simulink subsystem "Actuators_TVC_RCS"  (R2026a)
settings: Solver=VariableStepAuto
undefined symbols (not defined in the file): ENGINE, IN, VEH
libraries: simulink_extras x4, matrix_library x1
settings Model: Creator=asing  LastModifiedBy=asing

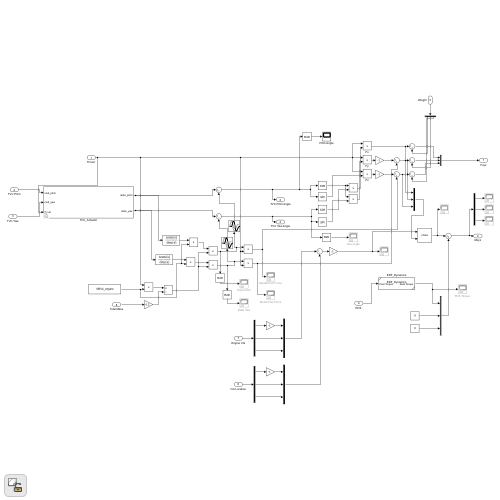
[thumbnail: Simulink's stored preview of the top-level diagram]
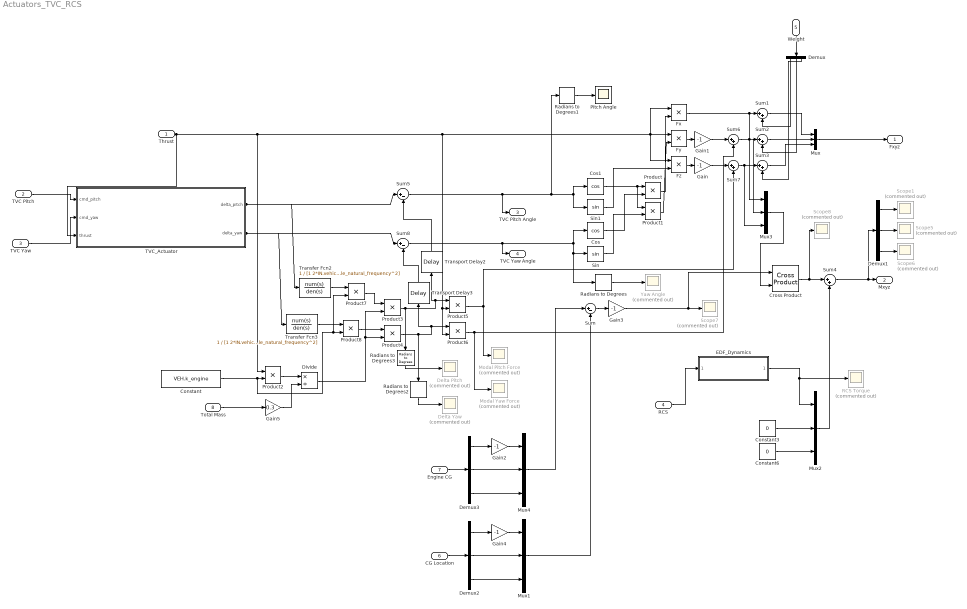
== system Actuators_TVC_RCS ==
  "Thrust " : Inport
  TVC Pitch : Inport  Port=2
  TVC Yaw : Inport  Port=3
  "RCS " : Inport  Port=4
  Weight : Inport  Port=5
  CG Location : Inport  Port=6
  Engine CG : Inport  Port=7
  Total Mass : Inport  Port=8
  Constant : Constant  Value=VEH.k_engine
  Constant3 : Constant  Value=0
  Constant6 : Constant  Value=0
  Cos : Trigonometry  Operator=cos
  Cos1 : Trigonometry  Operator=cos
  Cross Product : matrix_library/Cross Product
  Delta Pitch : Scope  Commented=on
      settings: ActiveDisplayYMinimum=-0.0038016775387335047  ActiveDisplayYMaximum=0.0038576393364572227  DataLoggingVariableName=ScopeData83
  Delta Yaw : Scope  Commented=on
      settings: ActiveDisplayYMinimum=-0.0018754271280055322  ActiveDisplayYMaximum=0.0029155281667496203  DataLoggingVariableName=ScopeData84
  Demux{,1..3} (4 alike) : Demux  Outputs=3
  Divide : Product  Inputs=*/
  EDF_Dynamics : Subsystem  ReferencedSubsystem=EDF_Dynamics
  Fx : Product
  Fy : Product
  Fz : Product
  Gain{,1..4} (5 alike) : Gain  Gain=-1
  Gain5 : Gain  Gain=0.3
  Modal Pitch Force : Scope  Commented=on
      settings: ActiveDisplayYMinimum=-0.088739631277941974  ActiveDisplayYMaximum=0.086025104693778914  DataLoggingVariableName=ScopeData78
  Modal Yaw Force : Scope  Commented=on
      settings: ActiveDisplayYMinimum=-0.017420268895536287  ActiveDisplayYMaximum=0.028077380315148965  DataLoggingVariableName=ScopeData79
  Mux{,1..4} (5 alike) : Mux  Inputs=3
  Pitch Angle : Scope
      settings: ActiveDisplayYMinimum=-10.903439073445846  ActiveDisplayYMaximum=7.4616563198748231  DataLoggingVariableName=ScopeData71
  Product{,1..8} (9 alike) : Product
  RCS Torque : Scope  Commented=on
      settings: ActiveDisplayYMinimum=-8.021209014289818  ActiveDisplayYMaximum=10.60123996530198  DataLoggingVariableName=ScopeData47
  Radians to Degrees{,1..3} (4 alike) : simulink_extras/Transformations/Radians to Degrees
  Scope{1,5..8} (5 alike) : Scope  Commented=on
      Scope1 settings: ActiveDisplayYMinimum=0.090000000000000011  ActiveDisplayYMaximum=0.11  DataLoggingVariableName=ScopeData50
      Scope5 settings: ActiveDisplayYMinimum=-1  ActiveDisplayYMaximum=1  DataLoggingVariableName=ScopeData54
      Scope6 settings: ActiveDisplayYMinimum=-1  ActiveDisplayYMaximum=1  DataLoggingVariableName=ScopeData55
      Scope7 settings: ActiveDisplayYMinimum=-1.008334185713273  ActiveDisplayYMaximum=-0.924758879501166  DataLoggingVariableName=ScopeData56
      Scope8 settings: ActiveDisplayYMinimum=-1  ActiveDisplayYMaximum=1  DataLoggingVariableName=ScopeData60
  Sin : Trigonometry
  Sin1 : Trigonometry
  Sum : Sum  Inputs=|+-
  Sum{1..4,6..7} (6 alike) : Sum  Inputs=|++
  Sum5 : Sum  Inputs=|+-
  Sum8 : Sum  Inputs=|+-
  TVC_Actuator : Subsystem  Variant=on
  Transfer Fcn2 : TransferFcn  Numerator=1  Denominator=[1 2*IN.vehicle_damping_ratio*IN.vehicle_natural_frequency IN.vehicle_natural_frequency^2]
  Transfer Fcn3 : TransferFcn  Numerator=1  Denominator=[1 2*IN.vehicle_damping_ratio*IN.vehicle_natural_frequency IN.vehicle_natural_frequency^2]
  Transport Delay2 : TransportDelay  DelayTime=0.01
  Transport Delay3 : TransportDelay  DelayTime=0.01
  Yaw Angle : Scope  Commented=on
      settings: ActiveDisplayYMinimum=-1.8231379337691429  ActiveDisplayYMaximum=5.2718467554145434  DataLoggingVariableName=ScopeData70
  Fxyz : Outport
  Mxyz : Outport  Port=2
  TVC Pitch Angle : Outport  Port=3
  TVC Yaw Angle : Outport  Port=4
  wires:
  Cos1/1 -> Product/1, Product1/1
  Cos/1 -> Product/2
  Product/1 -> Fx/2
  "Thrust "/1 -> Fz/1, Fy/1, Fx/1, Product5/2, Product6/2, Product2/1, TVC_Actuator/3(thrust)
  Mux/1 -> Fxyz/1
  Sum1/1 -> Mux/1
  Weight/1 -> Demux/1
  Fy/1 -> Gain1/1
  Sum2/1 -> Mux/2
  Fz/1 -> Gain/1
  Demux/2 -> Sum2/2
  Mux1/1 -> Sum/2
  Sum/1 -> Gain3/1
  Cross Product/1 -> Sum4/1, Scope8/1
  Constant3/1 -> Mux2/2
  Mux2/1 -> Sum4/2
  Sum4/1 -> Mxyz/1, Demux1/1
  Demux1/1 -> Scope1/1
  Demux1/2 -> Scope5/1
  Demux1/3 -> Scope6/1
  Product1/1 -> Fy/2
  Sin/1 -> Product1/2
  Sin1/1 -> Fz/2
  Gain3/1 -> Scope7/1, Cross Product/1
  Sum3/1 -> Mux/3
  Mux3/1 -> Cross Product/2
  Constant6/1 -> Mux2/3
  Demux/1 -> Sum1/2
  Demux/3 -> Sum3/2
  Radians to Degrees/1 -> Yaw Angle/1
  Radians to Degrees1/1 -> Pitch Angle/1
  "RCS "/1 -> EDF_Dynamics/1
  Demux2/3 -> Mux1/3
  CG Location/1 -> Demux2/1
  Demux2/2 -> Mux1/2
  Demux2/1 -> Gain4/1
  Gain4/1 -> Mux1/1
  Gain2/1 -> Mux4/1
  Demux3/1 -> Gain2/1
  Demux3/2 -> Mux4/2
  Demux3/3 -> Mux4/3
  Engine CG/1 -> Demux3/1
  Mux4/1 -> Sum/1
  Total Mass/1 -> Gain5/1
  Product2/1 -> Divide/1
  Gain5/1 -> Divide/2
  Constant/1 -> Product2/2, Product8/2, Product7/2
  Divide/1 -> Product4/2, Product3/2
  Product3/1 -> Radians to Degrees3/1, Product5/1, Transport Delay2/1
  Product4/1 -> Product6/1, Transport Delay3/1, Radians to Degrees2/1
  Fx/1 -> Sum1/1, Mux3/1
  Gain1/1 -> Sum6/1
  Sum6/1 -> Sum2/1, Mux3/2
  Gain/1 -> Sum7/1
  Sum7/1 -> Mux3/3, Sum3/1
  Product5/1 -> Modal Pitch Force/1, Sum7/2
  Product6/1 -> Modal Yaw Force/1, Sum6/2
  Sum5/1 -> Cos1/1, Sin1/1, Radians to Degrees1/1, TVC Pitch Angle/1
  Sum8/1 -> Cos/1, Radians to Degrees/1, Sin/1, TVC Yaw Angle/1
  Radians to Degrees2/1 -> Delta Yaw/1
  Radians to Degrees3/1 -> Delta Pitch/1
  Transport Delay3/1 -> Sum8/2
  Transport Delay2/1 -> Sum5/2
  Transfer Fcn2/1 -> Product7/1
  Product7/1 -> Product3/1
  Transfer Fcn3/1 -> Product8/1
  Product8/1 -> Product4/1
  EDF_Dynamics/1 -> RCS Torque/1, Mux2/1
  TVC Pitch/1 -> TVC_Actuator/1(cmd_pitch)
  TVC Yaw/1 -> TVC_Actuator/2(cmd_yaw)
  TVC_Actuator/1(delta_pitch) -> Sum5/1, Transfer Fcn2/1
  TVC_Actuator/2(delta_yaw) -> Sum8/1, Transfer Fcn3/1

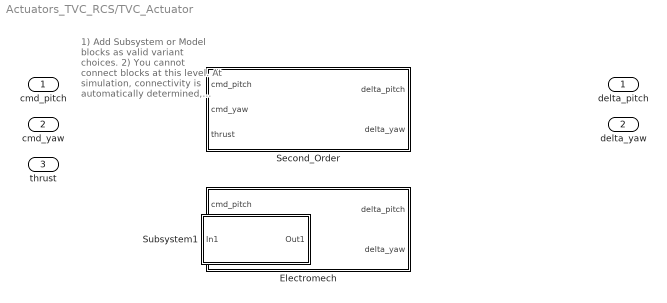
== system Actuators_TVC_RCS/TVC_Actuator ==
  note: 1) Add Subsystem or Model blocks as valid variant choices.
      | 2) You cannot connect blocks at this level. At simulation, connectivity is automatically
      | determined, based on the active variant and port name matching.
  cmd_pitch : Inport
  cmd_yaw : Inport  Port=2
  thrust : Inport  Port=3
  Electromech : Subsystem  VariantControl=VARIANT_TVC_MODEL >= 2
  Second_Order : Subsystem  VariantControl=VARIANT_TVC_MODEL == 1
  Subsystem1 : Subsystem  VariantControl=false
  delta_pitch : Outport
  delta_yaw : Outport  Port=2

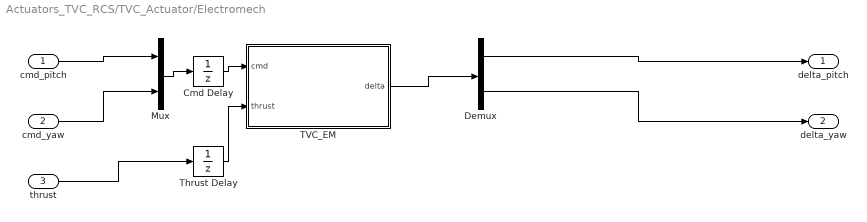
== system Actuators_TVC_RCS/TVC_Actuator/Electromech ==
  cmd_pitch : Inport
  cmd_yaw : Inport  Port=2
  thrust : Inport  Port=3
  Cmd Delay : UnitDelay  SampleTime=1e-3
  Demux : Demux  Outputs=2
  Mux : Mux  Inputs=2
  TVC_EM : MATLAB Function  TreatAsAtomicUnit=on
  Thrust Delay : UnitDelay  SampleTime=1e-3
  delta_pitch : Outport
  delta_yaw : Outport  Port=2
  wires:
  cmd_pitch/1 -> Mux/1
  cmd_yaw/1 -> Mux/2
  Mux/1 -> Cmd Delay/1
  Cmd Delay/1 -> TVC_EM/1(cmd)
  thrust/1 -> Thrust Delay/1
  Thrust Delay/1 -> TVC_EM/2(thrust)
  TVC_EM/1(delta) -> Demux/1
  Demux/1 -> delta_pitch/1
  Demux/2 -> delta_yaw/1

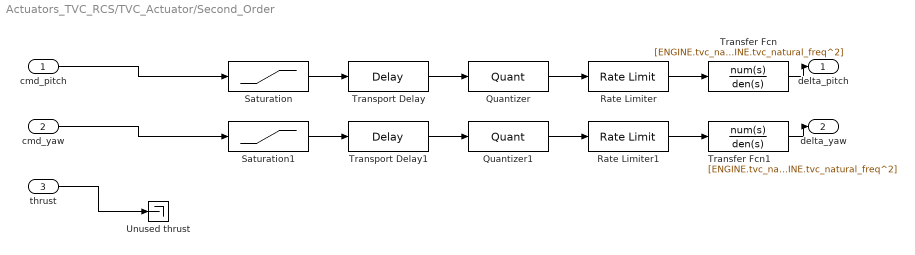
== system Actuators_TVC_RCS/TVC_Actuator/Second_Order ==
  cmd_pitch : Inport
  cmd_yaw : Inport  Port=2
  thrust : Inport  Port=3
  Quantizer : Quantizer  QuantizationInterval=IN.tvc.resolution
  Quantizer1 : Quantizer  QuantizationInterval=IN.tvc.resolution
  Rate Limiter : RateLimiter  RisingSlewLimit=IN.tvc.max_gimbal_rate  FallingSlewLimit=-IN.tvc.max_gimbal_rate  SampleTimeMode=inherited
  Rate Limiter1 : RateLimiter  RisingSlewLimit=IN.tvc.max_gimbal_rate  FallingSlewLimit=-IN.tvc.max_gimbal_rate  SampleTimeMode=inherited
  Saturation : Saturate  UpperLimit=IN.tvc.max_gimbal_angle  LowerLimit=-IN.tvc.max_gimbal_angle
  Saturation1 : Saturate  UpperLimit=IN.tvc.max_gimbal_angle  LowerLimit=-IN.tvc.max_gimbal_angle  LinearizeAsGain=off
  Transfer Fcn : TransferFcn  Numerator=[ENGINE.tvc_natural_freq^2]  Denominator=[1 2*IN.tvc.damping_ratio*ENGINE.tvc_natural_freq ENGINE.tvc_natural_freq^2]
  Transfer Fcn1 : TransferFcn  Numerator=[ENGINE.tvc_natural_freq^2]  Denominator=[1 2*IN.tvc.damping_ratio*ENGINE.tvc_natural_freq ENGINE.tvc_natural_freq^2]
  Transport Delay : TransportDelay  DelayTime=IN.tvc.actuator_latency
  Transport Delay1 : TransportDelay  DelayTime=IN.tvc.actuator_latency
  Unused thrust : Terminator
  delta_pitch : Outport
  delta_yaw : Outport  Port=2
  wires:
  cmd_pitch/1 -> Saturation/1
  Saturation/1 -> Transport Delay/1
  Transport Delay/1 -> Quantizer/1
  Quantizer/1 -> Rate Limiter/1
  Rate Limiter/1 -> Transfer Fcn/1
  Transfer Fcn/1 -> delta_pitch/1
  cmd_yaw/1 -> Saturation1/1
  Saturation1/1 -> Transport Delay1/1
  Transport Delay1/1 -> Quantizer1/1
  Quantizer1/1 -> Rate Limiter1/1
  Rate Limiter1/1 -> Transfer Fcn1/1
  Transfer Fcn1/1 -> delta_yaw/1
  thrust/1 -> Unused thrust/1

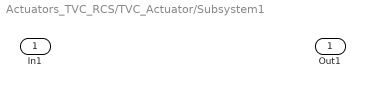
== system Actuators_TVC_RCS/TVC_Actuator/Subsystem1 ==
  In1 : Inport
  Out1 : Outport

== matlab function Actuators_TVC_RCS/TVC_Actuator/Electromech/TVC_EM ==
  data: cmd input; delta output size=[2 1]; thrust input; TVCEM parameter
function delta = TVC_EM(cmd, thrust, TVCEM)
% Erhardt+Leimer TVC actuators, voltage to gimbal angle (src/tvc/tvcEmUpdate.m),
% one call per 1 kHz servo period; cmd and delta are [pitch; yaw] in rad.
% (tools/refactor/addTvcModelVariant.m)
persistent S
if isempty(S), S = tvcEmInit(); end
[S, delta] = tvcEmUpdate(S, cmd, thrust, TVCEM);
end
